simulink model "Residential_grid5"  (R2026a)
settings: Solver=VariableStepAuto  StopTime=365*24*3600
undefined symbols (not defined in the file): evCharge, load1, load2, load3, load4, load5, Solar, Wind
libraries: fl_lib x139, nesl_utility x68
(part 1 of 3)
settings Model: Creator=xiaos  LastModifiedBy=hiro
settings DebuggingCC: SaveWithParameterizedLinksMsg=none
settings SimscapeCC: SimscapeNominalValues="[{\"value\":\"1\",\"unit\":\"A\"},{\"value\":\"1\",\"unit\":\"bar\"},{\"value\":\"1\",\"unit\":\"cm^2\"},{\"value\":\"1\",\"unit\":\"cm^3/s\"},{\"value\":\"1\",\"unit\":\"kJ/kg\"},{\"value\":\"1\",\"unit\":\"kW\"},{\"value\":\"1\",\"unit\":\"l\"},{\"value\":\"1\",\"unit\":\"N\"},{\"value\":\"1\",\"unit\":\"N*m\"},{\"value\":\"1\",\"unit\":\"V\"}]"  SimscapeLogType=none  SimscapeLogDataHistory=5000.0

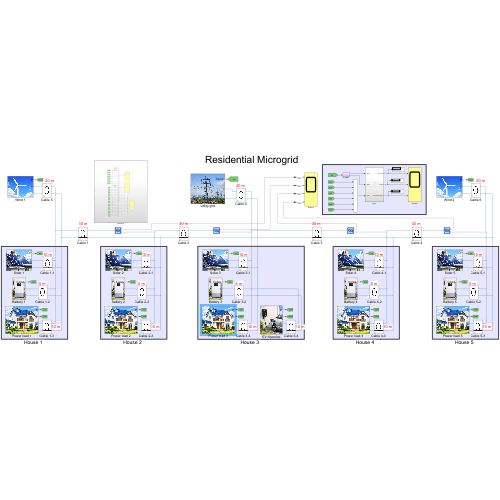
[thumbnail: Simulink's stored preview of the top-level diagram]
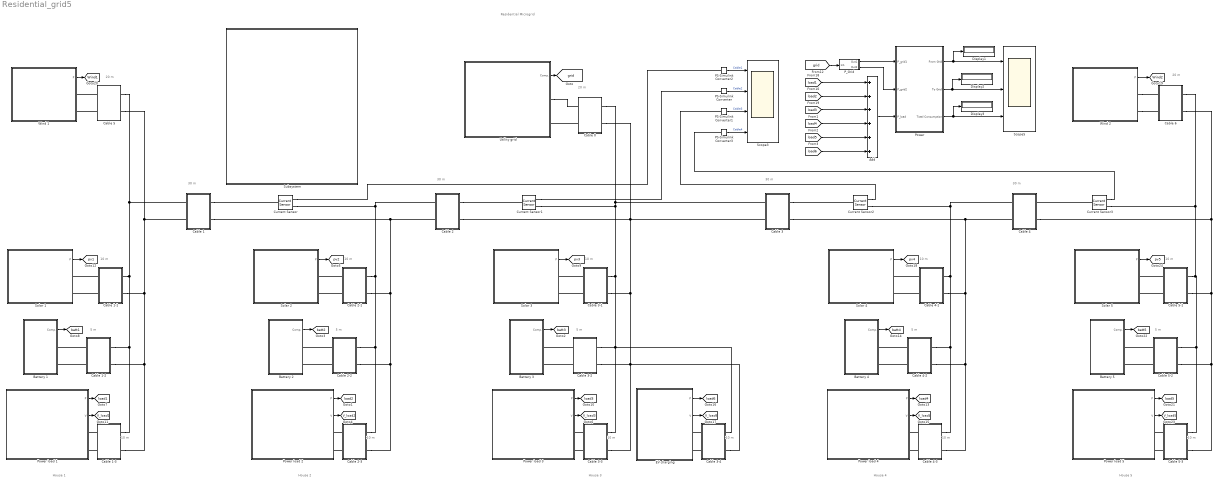
== system Residential_grid5 ==
  note: House 3
  note: House 2
  note: House 1
  note: House 4
  note: House 5
  note: Residential Microgrid
  note: 30 m
  note: 30 m
  note: 30 m
  note: 30 m
  note: 20 m
  note: 20 m
  note: 20 m
  note: 10 m
  note: 10 m
  note: 10 m
  note: 10 m
  note: 10 m
  note: 5 m
  note: 5 m
  note: 5 m
  note: 5 m
  note: 5 m
  note: 10 m
  note: 10 m
  note: 10 m
  note: 10 m
  note: 10 m
  note: 10 m
  Add : Sum  Inputs=++++++
  Battery 1 : Subsystem  mask{Cell=115, C_batt=20, SOC_Initial=50, R_int=75}
      mask prompts: Cell "Number of serial cells"; C_batt "Battery capacity (Ah)"; SOC_Initial "Initial SoC (%)"; R_int "Internal resistance (mΩ per Cell per Ah)"
      mask DialogControl DescTextVar Prompt: LiFePO4 Battery
      mask Display: image('Batt_1_4_1_1.png');
  Battery 2 : Subsystem  mask{Cell=115, C_batt=20, SOC_Initial=50, R_int=75}
      mask prompts: Cell "Number of serial cells"; C_batt "Battery capacity (Ah)"; SOC_Initial "Initial SoC (%)"; R_int "Internal resistance (mΩ per Cell per Ah)"
      mask DialogControl DescTextVar Prompt: LiFePO4 Battery
      mask Display: image('Batt_1_4_1_1.png');
  Battery 3 : Subsystem  mask{Cell=115, C_batt=20, SOC_Initial=50, R_int=75}
      mask prompts: Cell "Number of serial cells"; C_batt "Battery capacity (Ah)"; SOC_Initial "Initial SoC (%)"; R_int "Internal resistance (mΩ per Cell per Ah)"
      mask DialogControl DescTextVar Prompt: LiFePO4 Battery
      mask Display: image('Batt_1_4_1_1.png');
  Battery 4 : Subsystem  mask{Cell=115, C_batt=20, SOC_Initial=50, R_int=75}
      mask prompts: Cell "Number of serial cells"; C_batt "Battery capacity (Ah)"; SOC_Initial "Initial SoC (%)"; R_int "Internal resistance (mΩ per Cell per Ah)"
      mask DialogControl DescTextVar Prompt: LiFePO4 Battery
      mask Display: image('Batt_1_4_1_1.png');
  Battery 5 : Subsystem  mask{Cell=115, C_batt=20, SOC_Initial=50, R_int=75}
      mask prompts: Cell "Number of serial cells"; C_batt "Battery capacity (Ah)"; SOC_Initial "Initial SoC (%)"; R_int "Internal resistance (mΩ per Cell per Ah)"
      mask DialogControl DescTextVar Prompt: LiFePO4 Battery
      mask Display: image('Batt_1_4_1_1.png');
  Cable 0 : Subsystem  mask{intR=3.01, L=20, SQ=SQ,  rc,  Ampacity}
      mask prompts: intR "Conductor resistance: rc (Ω/km)"; L "Length: L (m)"; SQ "For reference: CV cable constants"
      mask TypeOptions SQ: SQ,  rc,  Ampacity | 2 (mm2),  12 (Ω/km),  28 (A) | 3.5 (mm2),  6.76 (Ω/km),  39 (A) | 5.5 (mm2),  4.34 (Ω/km),  52 (A) | 8 (mm2),  3.01 (Ω/km),   65 (A) | 14 (mm2),  1.71 (Ω/km),  91 (A) | 22 (mm2),  1.08 (Ω/km),  120 (A) | 38 (mm2),  0.626 (Ω/km),  170 (A) | 60 (mm2),  0.397 (Ω/km),  225 (A) | 100 (mm2),  0.239 (Ω/km),  310 (A) | 150 (mm2),  0.16 (Ω/km),  400 (A) | 200 (mm2),  0.121 (Ω/km),  485 (A) | 250 (mm2),  0.0985 (Ω/km),  560 (A) | 325 (mm2),  0.077 (Ω/km),  660 (A)
      mask DialogControl DescTextVar Prompt: 2-Core CV Cable
      mask Display: image('cable_1.png');
  Cable 1 : Subsystem  mask{intR=3.01, L=30, SQ=SQ,  rc,  Ampacity}
      mask prompts: intR "Conductor resistance: rc (Ω/km)"; L "Length: L (m)"; SQ "For reference: CV cable constants"
      mask TypeOptions SQ: SQ,  rc,  Ampacity | 2 (mm2),  12 (Ω/km),  28 (A) | 3.5 (mm2),  6.76 (Ω/km),  39 (A) | 5.5 (mm2),  4.34 (Ω/km),  52 (A) | 8 (mm2),  3.01 (Ω/km),   65 (A) | 14 (mm2),  1.71 (Ω/km),  91 (A) | 22 (mm2),  1.08 (Ω/km),  120 (A) | 38 (mm2),  0.626 (Ω/km),  170 (A) | 60 (mm2),  0.397 (Ω/km),  225 (A) | 100 (mm2),  0.239 (Ω/km),  310 (A) | 150 (mm2),  0.16 (Ω/km),  400 (A) | 200 (mm2),  0.121 (Ω/km),  485 (A) | 250 (mm2),  0.0985 (Ω/km),  560 (A) | 325 (mm2),  0.077 (Ω/km),  660 (A)
      mask DialogControl DescTextVar Prompt: 2-Core CV Cable
      mask Display: image('cable_2.png');
  Cable 1-1 : Subsystem  mask{intR=3.01, L=10, SQ=SQ,  rc,  Ampacity}
      mask prompts: intR "Conductor resistance: rc (Ω/km)"; L "Length: L (m)"; SQ "For reference: CV cable constants"
      mask TypeOptions SQ: SQ,  rc,  Ampacity | 2 (mm2),  12 (Ω/km),  28 (A) | 3.5 (mm2),  6.76 (Ω/km),  39 (A) | 5.5 (mm2),  4.34 (Ω/km),  52 (A) | 8 (mm2),  3.01 (Ω/km),   65 (A) | 14 (mm2),  1.71 (Ω/km),  91 (A) | 22 (mm2),  1.08 (Ω/km),  120 (A) | 38 (mm2),  0.626 (Ω/km),  170 (A) | 60 (mm2),  0.397 (Ω/km),  225 (A) | 100 (mm2),  0.239 (Ω/km),  310 (A) | 150 (mm2),  0.16 (Ω/km),  400 (A) | 200 (mm2),  0.121 (Ω/km),  485 (A) | 250 (mm2),  0.0985 (Ω/km),  560 (A) | 325 (mm2),  0.077 (Ω/km),  660 (A)
      mask DialogControl DescTextVar Prompt: 2-Core CV Cable
      mask Display: image('cable_9.png');
  Cable 1-2 : Subsystem  mask{intR=3.01, L=5, SQ=SQ,  rc,  Ampacity}
      mask prompts: intR "Conductor resistance: rc (Ω/km)"; L "Length: L (m)"; SQ "For reference: CV cable constants"
      mask TypeOptions SQ: SQ,  rc,  Ampacity | 2 (mm2),  12 (Ω/km),  28 (A) | 3.5 (mm2),  6.76 (Ω/km),  39 (A) | 5.5 (mm2),  4.34 (Ω/km),  52 (A) | 8 (mm2),  3.01 (Ω/km),   65 (A) | 14 (mm2),  1.71 (Ω/km),  91 (A) | 22 (mm2),  1.08 (Ω/km),  120 (A) | 38 (mm2),  0.626 (Ω/km),  170 (A) | 60 (mm2),  0.397 (Ω/km),  225 (A) | 100 (mm2),  0.239 (Ω/km),  310 (A) | 150 (mm2),  0.16 (Ω/km),  400 (A) | 200 (mm2),  0.121 (Ω/km),  485 (A) | 250 (mm2),  0.0985 (Ω/km),  560 (A) | 325 (mm2),  0.077 (Ω/km),  660 (A)
      mask DialogControl DescTextVar Prompt: 2-Core CV Cable
      mask Display: image('cable_7.png');
  Cable 1-3 : Subsystem  mask{intR=3.01, L=10, SQ=SQ,  rc,  Ampacity}
      mask prompts: intR "Conductor resistance: rc (Ω/km)"; L "Length: L (m)"; SQ "For reference: CV cable constants"
      mask TypeOptions SQ: SQ,  rc,  Ampacity | 2 (mm2),  12 (Ω/km),  28 (A) | 3.5 (mm2),  6.76 (Ω/km),  39 (A) | 5.5 (mm2),  4.34 (Ω/km),  52 (A) | 8 (mm2),  3.01 (Ω/km),   65 (A) | 14 (mm2),  1.71 (Ω/km),  91 (A) | 22 (mm2),  1.08 (Ω/km),  120 (A) | 38 (mm2),  0.626 (Ω/km),  170 (A) | 60 (mm2),  0.397 (Ω/km),  225 (A) | 100 (mm2),  0.239 (Ω/km),  310 (A) | 150 (mm2),  0.16 (Ω/km),  400 (A) | 200 (mm2),  0.121 (Ω/km),  485 (A) | 250 (mm2),  0.0985 (Ω/km),  560 (A) | 325 (mm2),  0.077 (Ω/km),  660 (A)
      mask DialogControl DescTextVar Prompt: 2-Core CV Cable
      mask Display: image('cable_8.png');
  Cable 2 : Subsystem  mask{intR=3.01, L=30, SQ=SQ,  rc,  Ampacity}
      mask prompts: intR "Conductor resistance: rc (Ω/km)"; L "Length: L (m)"; SQ "For reference: CV cable constants"
      mask TypeOptions SQ: SQ,  rc,  Ampacity | 2 (mm2),  12 (Ω/km),  28 (A) | 3.5 (mm2),  6.76 (Ω/km),  39 (A) | 5.5 (mm2),  4.34 (Ω/km),  52 (A) | 8 (mm2),  3.01 (Ω/km),   65 (A) | 14 (mm2),  1.71 (Ω/km),  91 (A) | 22 (mm2),  1.08 (Ω/km),  120 (A) | 38 (mm2),  0.626 (Ω/km),  170 (A) | 60 (mm2),  0.397 (Ω/km),  225 (A) | 100 (mm2),  0.239 (Ω/km),  310 (A) | 150 (mm2),  0.16 (Ω/km),  400 (A) | 200 (mm2),  0.121 (Ω/km),  485 (A) | 250 (mm2),  0.0985 (Ω/km),  560 (A) | 325 (mm2),  0.077 (Ω/km),  660 (A)
      mask DialogControl DescTextVar Prompt: 2-Core CV Cable
      mask Display: image('cable_3.png');
  Cable 2-1 : Subsystem  mask{intR=3.01, L=10, SQ=SQ,  rc,  Ampacity}
      mask prompts: intR "Conductor resistance: rc (Ω/km)"; L "Length: L (m)"; SQ "For reference: CV cable constants"
      mask TypeOptions SQ: SQ,  rc,  Ampacity | 2 (mm2),  12 (Ω/km),  28 (A) | 3.5 (mm2),  6.76 (Ω/km),  39 (A) | 5.5 (mm2),  4.34 (Ω/km),  52 (A) | 8 (mm2),  3.01 (Ω/km),   65 (A) | 14 (mm2),  1.71 (Ω/km),  91 (A) | 22 (mm2),  1.08 (Ω/km),  120 (A) | 38 (mm2),  0.626 (Ω/km),  170 (A) | 60 (mm2),  0.397 (Ω/km),  225 (A) | 100 (mm2),  0.239 (Ω/km),  310 (A) | 150 (mm2),  0.16 (Ω/km),  400 (A) | 200 (mm2),  0.121 (Ω/km),  485 (A) | 250 (mm2),  0.0985 (Ω/km),  560 (A) | 325 (mm2),  0.077 (Ω/km),  660 (A)
      mask DialogControl DescTextVar Prompt: 2-Core CV Cable
      mask Display: image('cable_9.png');
  Cable 2-2 : Subsystem  mask{intR=3.01, L=5, SQ=SQ,  rc,  Ampacity}
      mask prompts: intR "Conductor resistance: rc (Ω/km)"; L "Length: L (m)"; SQ "For reference: CV cable constants"
      mask TypeOptions SQ: SQ,  rc,  Ampacity | 2 (mm2),  12 (Ω/km),  28 (A) | 3.5 (mm2),  6.76 (Ω/km),  39 (A) | 5.5 (mm2),  4.34 (Ω/km),  52 (A) | 8 (mm2),  3.01 (Ω/km),   65 (A) | 14 (mm2),  1.71 (Ω/km),  91 (A) | 22 (mm2),  1.08 (Ω/km),  120 (A) | 38 (mm2),  0.626 (Ω/km),  170 (A) | 60 (mm2),  0.397 (Ω/km),  225 (A) | 100 (mm2),  0.239 (Ω/km),  310 (A) | 150 (mm2),  0.16 (Ω/km),  400 (A) | 200 (mm2),  0.121 (Ω/km),  485 (A) | 250 (mm2),  0.0985 (Ω/km),  560 (A) | 325 (mm2),  0.077 (Ω/km),  660 (A)
      mask DialogControl DescTextVar Prompt: 2-Core CV Cable
      mask Display: image('cable_7.png');
  Cable 2-3 : Subsystem  mask{intR=3.01, L=10, SQ=SQ,  rc,  Ampacity}
      mask prompts: intR "Conductor resistance: rc (Ω/km)"; L "Length: L (m)"; SQ "For reference: CV cable constants"
      mask TypeOptions SQ: SQ,  rc,  Ampacity | 2 (mm2),  12 (Ω/km),  28 (A) | 3.5 (mm2),  6.76 (Ω/km),  39 (A) | 5.5 (mm2),  4.34 (Ω/km),  52 (A) | 8 (mm2),  3.01 (Ω/km),   65 (A) | 14 (mm2),  1.71 (Ω/km),  91 (A) | 22 (mm2),  1.08 (Ω/km),  120 (A) | 38 (mm2),  0.626 (Ω/km),  170 (A) | 60 (mm2),  0.397 (Ω/km),  225 (A) | 100 (mm2),  0.239 (Ω/km),  310 (A) | 150 (mm2),  0.16 (Ω/km),  400 (A) | 200 (mm2),  0.121 (Ω/km),  485 (A) | 250 (mm2),  0.0985 (Ω/km),  560 (A) | 325 (mm2),  0.077 (Ω/km),  660 (A)
      mask DialogControl DescTextVar Prompt: 2-Core CV Cable
      mask Display: image('cable_8.png');
  Cable 3 : Subsystem  mask{intR=3.01, L=30, SQ=SQ,  rc,  Ampacity}
      mask prompts: intR "Conductor resistance: rc (Ω/km)"; L "Length: L (m)"; SQ "For reference: CV cable constants"
      mask TypeOptions SQ: SQ,  rc,  Ampacity | 2 (mm2),  12 (Ω/km),  28 (A) | 3.5 (mm2),  6.76 (Ω/km),  39 (A) | 5.5 (mm2),  4.34 (Ω/km),  52 (A) | 8 (mm2),  3.01 (Ω/km),   65 (A) | 14 (mm2),  1.71 (Ω/km),  91 (A) | 22 (mm2),  1.08 (Ω/km),  120 (A) | 38 (mm2),  0.626 (Ω/km),  170 (A) | 60 (mm2),  0.397 (Ω/km),  225 (A) | 100 (mm2),  0.239 (Ω/km),  310 (A) | 150 (mm2),  0.16 (Ω/km),  400 (A) | 200 (mm2),  0.121 (Ω/km),  485 (A) | 250 (mm2),  0.0985 (Ω/km),  560 (A) | 325 (mm2),  0.077 (Ω/km),  660 (A)
      mask DialogControl DescTextVar Prompt: 2-Core CV Cable
      mask Display: image('cable_4.png');
  Cable 3-1 : Subsystem  mask{intR=3.01, L=10, SQ=SQ,  rc,  Ampacity}
      mask prompts: intR "Conductor resistance: rc (Ω/km)"; L "Length: L (m)"; SQ "For reference: CV cable constants"
      mask TypeOptions SQ: SQ,  rc,  Ampacity | 2 (mm2),  12 (Ω/km),  28 (A) | 3.5 (mm2),  6.76 (Ω/km),  39 (A) | 5.5 (mm2),  4.34 (Ω/km),  52 (A) | 8 (mm2),  3.01 (Ω/km),   65 (A) | 14 (mm2),  1.71 (Ω/km),  91 (A) | 22 (mm2),  1.08 (Ω/km),  120 (A) | 38 (mm2),  0.626 (Ω/km),  170 (A) | 60 (mm2),  0.397 (Ω/km),  225 (A) | 100 (mm2),  0.239 (Ω/km),  310 (A) | 150 (mm2),  0.16 (Ω/km),  400 (A) | 200 (mm2),  0.121 (Ω/km),  485 (A) | 250 (mm2),  0.0985 (Ω/km),  560 (A) | 325 (mm2),  0.077 (Ω/km),  660 (A)
      mask DialogControl DescTextVar Prompt: 2-Core CV Cable
      mask Display: image('cable_9.png');
  Cable 3-2 : Subsystem  mask{intR=3.01, L=5, SQ=SQ,  rc,  Ampacity}
      mask prompts: intR "Conductor resistance: rc (Ω/km)"; L "Length: L (m)"; SQ "For reference: CV cable constants"
      mask TypeOptions SQ: SQ,  rc,  Ampacity | 2 (mm2),  12 (Ω/km),  28 (A) | 3.5 (mm2),  6.76 (Ω/km),  39 (A) | 5.5 (mm2),  4.34 (Ω/km),  52 (A) | 8 (mm2),  3.01 (Ω/km),   65 (A) | 14 (mm2),  1.71 (Ω/km),  91 (A) | 22 (mm2),  1.08 (Ω/km),  120 (A) | 38 (mm2),  0.626 (Ω/km),  170 (A) | 60 (mm2),  0.397 (Ω/km),  225 (A) | 100 (mm2),  0.239 (Ω/km),  310 (A) | 150 (mm2),  0.16 (Ω/km),  400 (A) | 200 (mm2),  0.121 (Ω/km),  485 (A) | 250 (mm2),  0.0985 (Ω/km),  560 (A) | 325 (mm2),  0.077 (Ω/km),  660 (A)
      mask DialogControl DescTextVar Prompt: 2-Core CV Cable
      mask Display: image('cable_7.png');
  Cable 3-3 : Subsystem  mask{intR=3.01, L=10, SQ=SQ,  rc,  Ampacity}
      mask prompts: intR "Conductor resistance: rc (Ω/km)"; L "Length: L (m)"; SQ "For reference: CV cable constants"
      mask TypeOptions SQ: SQ,  rc,  Ampacity | 2 (mm2),  12 (Ω/km),  28 (A) | 3.5 (mm2),  6.76 (Ω/km),  39 (A) | 5.5 (mm2),  4.34 (Ω/km),  52 (A) | 8 (mm2),  3.01 (Ω/km),   65 (A) | 14 (mm2),  1.71 (Ω/km),  91 (A) | 22 (mm2),  1.08 (Ω/km),  120 (A) | 38 (mm2),  0.626 (Ω/km),  170 (A) | 60 (mm2),  0.397 (Ω/km),  225 (A) | 100 (mm2),  0.239 (Ω/km),  310 (A) | 150 (mm2),  0.16 (Ω/km),  400 (A) | 200 (mm2),  0.121 (Ω/km),  485 (A) | 250 (mm2),  0.0985 (Ω/km),  560 (A) | 325 (mm2),  0.077 (Ω/km),  660 (A)
      mask DialogControl DescTextVar Prompt: 2-Core CV Cable
      mask Display: image('cable_8.png');
  Cable 3-4 : Subsystem  mask{intR=3.01, L=10, SQ=SQ,  rc,  Ampacity}
      mask prompts: intR "Conductor resistance: rc (Ω/km)"; L "Length: L (m)"; SQ "For reference: CV cable constants"
      mask TypeOptions SQ: SQ,  rc,  Ampacity | 2 (mm2),  12 (Ω/km),  28 (A) | 3.5 (mm2),  6.76 (Ω/km),  39 (A) | 5.5 (mm2),  4.34 (Ω/km),  52 (A) | 8 (mm2),  3.01 (Ω/km),   65 (A) | 14 (mm2),  1.71 (Ω/km),  91 (A) | 22 (mm2),  1.08 (Ω/km),  120 (A) | 38 (mm2),  0.626 (Ω/km),  170 (A) | 60 (mm2),  0.397 (Ω/km),  225 (A) | 100 (mm2),  0.239 (Ω/km),  310 (A) | 150 (mm2),  0.16 (Ω/km),  400 (A) | 200 (mm2),  0.121 (Ω/km),  485 (A) | 250 (mm2),  0.0985 (Ω/km),  560 (A) | 325 (mm2),  0.077 (Ω/km),  660 (A)
      mask DialogControl DescTextVar Prompt: 2-Core CV Cable
      mask Display: image('cable_8.png');
  Cable 4 : Subsystem  mask{intR=3.01, L=30, SQ=SQ,  rc,  Ampacity}
      mask prompts: intR "Conductor resistance: rc (Ω/km)"; L "Length: L (m)"; SQ "For reference: CV cable constants"
      mask TypeOptions SQ: SQ,  rc,  Ampacity | 2 (mm2),  12 (Ω/km),  28 (A) | 3.5 (mm2),  6.76 (Ω/km),  39 (A) | 5.5 (mm2),  4.34 (Ω/km),  52 (A) | 8 (mm2),  3.01 (Ω/km),   65 (A) | 14 (mm2),  1.71 (Ω/km),  91 (A) | 22 (mm2),  1.08 (Ω/km),  120 (A) | 38 (mm2),  0.626 (Ω/km),  170 (A) | 60 (mm2),  0.397 (Ω/km),  225 (A) | 100 (mm2),  0.239 (Ω/km),  310 (A) | 150 (mm2),  0.16 (Ω/km),  400 (A) | 200 (mm2),  0.121 (Ω/km),  485 (A) | 250 (mm2),  0.0985 (Ω/km),  560 (A) | 325 (mm2),  0.077 (Ω/km),  660 (A)
      mask DialogControl DescTextVar Prompt: 2-Core CV Cable
      mask Display: image('cable_5.png');
  Cable 4-1 : Subsystem  mask{intR=3.01, L=10, SQ=SQ,  rc,  Ampacity}
      mask prompts: intR "Conductor resistance: rc (Ω/km)"; L "Length: L (m)"; SQ "For reference: CV cable constants"
      mask TypeOptions SQ: SQ,  rc,  Ampacity | 2 (mm2),  12 (Ω/km),  28 (A) | 3.5 (mm2),  6.76 (Ω/km),  39 (A) | 5.5 (mm2),  4.34 (Ω/km),  52 (A) | 8 (mm2),  3.01 (Ω/km),   65 (A) | 14 (mm2),  1.71 (Ω/km),  91 (A) | 22 (mm2),  1.08 (Ω/km),  120 (A) | 38 (mm2),  0.626 (Ω/km),  170 (A) | 60 (mm2),  0.397 (Ω/km),  225 (A) | 100 (mm2),  0.239 (Ω/km),  310 (A) | 150 (mm2),  0.16 (Ω/km),  400 (A) | 200 (mm2),  0.121 (Ω/km),  485 (A) | 250 (mm2),  0.0985 (Ω/km),  560 (A) | 325 (mm2),  0.077 (Ω/km),  660 (A)
      mask DialogControl DescTextVar Prompt: 2-Core CV Cable
      mask Display: image('cable_9.png');
  Cable 4-2 : Subsystem  mask{intR=3.01, L=5, SQ=SQ,  rc,  Ampacity}
      mask prompts: intR "Conductor resistance: rc (Ω/km)"; L "Length: L (m)"; SQ "For reference: CV cable constants"
      mask TypeOptions SQ: SQ,  rc,  Ampacity | 2 (mm2),  12 (Ω/km),  28 (A) | 3.5 (mm2),  6.76 (Ω/km),  39 (A) | 5.5 (mm2),  4.34 (Ω/km),  52 (A) | 8 (mm2),  3.01 (Ω/km),   65 (A) | 14 (mm2),  1.71 (Ω/km),  91 (A) | 22 (mm2),  1.08 (Ω/km),  120 (A) | 38 (mm2),  0.626 (Ω/km),  170 (A) | 60 (mm2),  0.397 (Ω/km),  225 (A) | 100 (mm2),  0.239 (Ω/km),  310 (A) | 150 (mm2),  0.16 (Ω/km),  400 (A) | 200 (mm2),  0.121 (Ω/km),  485 (A) | 250 (mm2),  0.0985 (Ω/km),  560 (A) | 325 (mm2),  0.077 (Ω/km),  660 (A)
      mask DialogControl DescTextVar Prompt: 2-Core CV Cable
      mask Display: image('cable_7.png');
  Cable 4-3 : Subsystem  mask{intR=3.01, L=10, SQ=SQ,  rc,  Ampacity}
      mask prompts: intR "Conductor resistance: rc (Ω/km)"; L "Length: L (m)"; SQ "For reference: CV cable constants"
      mask TypeOptions SQ: SQ,  rc,  Ampacity | 2 (mm2),  12 (Ω/km),  28 (A) | 3.5 (mm2),  6.76 (Ω/km),  39 (A) | 5.5 (mm2),  4.34 (Ω/km),  52 (A) | 8 (mm2),  3.01 (Ω/km),   65 (A) | 14 (mm2),  1.71 (Ω/km),  91 (A) | 22 (mm2),  1.08 (Ω/km),  120 (A) | 38 (mm2),  0.626 (Ω/km),  170 (A) | 60 (mm2),  0.397 (Ω/km),  225 (A) | 100 (mm2),  0.239 (Ω/km),  310 (A) | 150 (mm2),  0.16 (Ω/km),  400 (A) | 200 (mm2),  0.121 (Ω/km),  485 (A) | 250 (mm2),  0.0985 (Ω/km),  560 (A) | 325 (mm2),  0.077 (Ω/km),  660 (A)
      mask DialogControl DescTextVar Prompt: 2-Core CV Cable
      mask Display: image('cable_8.png');
  Cable 5 : Subsystem  mask{intR=3.01, L=20, SQ=SQ,  rc,  Ampacity}
      mask prompts: intR "Conductor resistance: rc (Ω/km)"; L "Length: L (m)"; SQ "For reference: CV cable constants"
      mask TypeOptions SQ: SQ,  rc,  Ampacity | 2 (mm2),  12 (Ω/km),  28 (A) | 3.5 (mm2),  6.76 (Ω/km),  39 (A) | 5.5 (mm2),  4.34 (Ω/km),  52 (A) | 8 (mm2),  3.01 (Ω/km),   65 (A) | 14 (mm2),  1.71 (Ω/km),  91 (A) | 22 (mm2),  1.08 (Ω/km),  120 (A) | 38 (mm2),  0.626 (Ω/km),  170 (A) | 60 (mm2),  0.397 (Ω/km),  225 (A) | 100 (mm2),  0.239 (Ω/km),  310 (A) | 150 (mm2),  0.16 (Ω/km),  400 (A) | 200 (mm2),  0.121 (Ω/km),  485 (A) | 250 (mm2),  0.0985 (Ω/km),  560 (A) | 325 (mm2),  0.077 (Ω/km),  660 (A)
      mask DialogControl DescTextVar Prompt: 2-Core CV Cable
      mask Display: image('cable_6.png');
  Cable 5-1 : Subsystem  mask{intR=3.01, L=10, SQ=SQ,  rc,  Ampacity}
      mask prompts: intR "Conductor resistance: rc (Ω/km)"; L "Length: L (m)"; SQ "For reference: CV cable constants"
      mask TypeOptions SQ: SQ,  rc,  Ampacity | 2 (mm2),  12 (Ω/km),  28 (A) | 3.5 (mm2),  6.76 (Ω/km),  39 (A) | 5.5 (mm2),  4.34 (Ω/km),  52 (A) | 8 (mm2),  3.01 (Ω/km),   65 (A) | 14 (mm2),  1.71 (Ω/km),  91 (A) | 22 (mm2),  1.08 (Ω/km),  120 (A) | 38 (mm2),  0.626 (Ω/km),  170 (A) | 60 (mm2),  0.397 (Ω/km),  225 (A) | 100 (mm2),  0.239 (Ω/km),  310 (A) | 150 (mm2),  0.16 (Ω/km),  400 (A) | 200 (mm2),  0.121 (Ω/km),  485 (A) | 250 (mm2),  0.0985 (Ω/km),  560 (A) | 325 (mm2),  0.077 (Ω/km),  660 (A)
      mask DialogControl DescTextVar Prompt: 2-Core CV Cable
      mask Display: image('cable_9.png');
  Cable 5-2 : Subsystem  mask{intR=3.01, L=5, SQ=SQ,  rc,  Ampacity}
      mask prompts: intR "Conductor resistance: rc (Ω/km)"; L "Length: L (m)"; SQ "For reference: CV cable constants"
      mask TypeOptions SQ: SQ,  rc,  Ampacity | 2 (mm2),  12 (Ω/km),  28 (A) | 3.5 (mm2),  6.76 (Ω/km),  39 (A) | 5.5 (mm2),  4.34 (Ω/km),  52 (A) | 8 (mm2),  3.01 (Ω/km),   65 (A) | 14 (mm2),  1.71 (Ω/km),  91 (A) | 22 (mm2),  1.08 (Ω/km),  120 (A) | 38 (mm2),  0.626 (Ω/km),  170 (A) | 60 (mm2),  0.397 (Ω/km),  225 (A) | 100 (mm2),  0.239 (Ω/km),  310 (A) | 150 (mm2),  0.16 (Ω/km),  400 (A) | 200 (mm2),  0.121 (Ω/km),  485 (A) | 250 (mm2),  0.0985 (Ω/km),  560 (A) | 325 (mm2),  0.077 (Ω/km),  660 (A)
      mask DialogControl DescTextVar Prompt: 2-Core CV Cable
      mask Display: image('cable_7.png');
  Cable 5-3 : Subsystem  mask{intR=3.01, L=10, SQ=SQ,  rc,  Ampacity}
      mask prompts: intR "Conductor resistance: rc (Ω/km)"; L "Length: L (m)"; SQ "For reference: CV cable constants"
      mask TypeOptions SQ: SQ,  rc,  Ampacity | 2 (mm2),  12 (Ω/km),  28 (A) | 3.5 (mm2),  6.76 (Ω/km),  39 (A) | 5.5 (mm2),  4.34 (Ω/km),  52 (A) | 8 (mm2),  3.01 (Ω/km),   65 (A) | 14 (mm2),  1.71 (Ω/km),  91 (A) | 22 (mm2),  1.08 (Ω/km),  120 (A) | 38 (mm2),  0.626 (Ω/km),  170 (A) | 60 (mm2),  0.397 (Ω/km),  225 (A) | 100 (mm2),  0.239 (Ω/km),  310 (A) | 150 (mm2),  0.16 (Ω/km),  400 (A) | 200 (mm2),  0.121 (Ω/km),  485 (A) | 250 (mm2),  0.0985 (Ω/km),  560 (A) | 325 (mm2),  0.077 (Ω/km),  660 (A)
      mask DialogControl DescTextVar Prompt: 2-Core CV Cable
      mask Display: image('cable_8.png');
  Cable 6 : Subsystem  mask{intR=3.01, L=20, SQ=SQ,  rc,  Ampacity}
      mask prompts: intR "Conductor resistance: rc (Ω/km)"; L "Length: L (m)"; SQ "For reference: CV cable constants"
      mask TypeOptions SQ: SQ,  rc,  Ampacity | 2 (mm2),  12 (Ω/km),  28 (A) | 3.5 (mm2),  6.76 (Ω/km),  39 (A) | 5.5 (mm2),  4.34 (Ω/km),  52 (A) | 8 (mm2),  3.01 (Ω/km),   65 (A) | 14 (mm2),  1.71 (Ω/km),  91 (A) | 22 (mm2),  1.08 (Ω/km),  120 (A) | 38 (mm2),  0.626 (Ω/km),  170 (A) | 60 (mm2),  0.397 (Ω/km),  225 (A) | 100 (mm2),  0.239 (Ω/km),  310 (A) | 150 (mm2),  0.16 (Ω/km),  400 (A) | 200 (mm2),  0.121 (Ω/km),  485 (A) | 250 (mm2),  0.0985 (Ω/km),  560 (A) | 325 (mm2),  0.077 (Ω/km),  660 (A)
      mask DialogControl DescTextVar Prompt: 2-Core CV Cable
      mask Display: image('cable_6.png');
  Current Sensor{,1..3} (4 alike) : fl_lib/Electrical/Electrical Sensors/Current Sensor
  Display1 : Display
  Display2 : Display
  Display3 : Display
  EV charging : Subsystem  mask{data=evCharge, timestep=[0:1:24*3600*365-1]}
      mask prompts: data "Power consumption data"
      mask DialogControl DescGroupVar Prompt: EV Charging
      mask Display: image('EV_Charge_1.png');
  PS-Simulink Converter{,1..3} (4 alike) : nesl_utility/PS-Simulink Converter  PhysicalDomain=network_engine_domain  SubClassName=ps_output  LeftPortType=input  RightPortType=output  PseudoPeriodic=off  Frequencies=[]  VectorFormat=inherit  Unit=inherit  AffineConversion=off
  P_Grid : Subsystem
  Power : Subsystem
  Power load 1 : Subsystem  mask{data=load1, timestep=[0:1:24*3600*365-1]}
      mask prompts: data "Power consumption data"
      mask DialogControl DescGroupVar Prompt: Power Load
      mask Display: image('House_1.png');
  Power load 2 : Subsystem  mask{data=load2, timestep=[0:1:24*3600*365-1]}
      mask prompts: data "Power consumption data"
      mask DialogControl DescGroupVar Prompt: Power Load
      mask Display: image('House_1.png');
  Power load 3 : Subsystem  mask{data=load3, timestep=[0:1:24*3600*365-1]}
      mask prompts: data "Power consumption data"
      mask DialogControl DescGroupVar Prompt: Power Load
      mask Display: image('House_1.png');
  Power load 4 : Subsystem  mask{data=load4, timestep=[0:1:24*3600*365-1]}
      mask prompts: data "Power consumption data"
      mask DialogControl DescGroupVar Prompt: Power Load
      mask Display: image('House_1.png');
  Power load 5 : Subsystem  mask{data=load5, timestep=[0:1:24*3600*365-1]}
      mask prompts: data "Power consumption data"
      mask DialogControl DescGroupVar Prompt: Power Load
      mask Display: image('House_1.png');
  Scope3 : Scope  NumInputPorts=4
      settings: ActiveDisplayYMinimum=-18.216451642812157  ActiveDisplayYMaximum=17.414891932696229  YLabel=Current (A)  DataLoggingDecimation=60
  Scope5 : Scope  NumInputPorts=3
      settings: ActiveDisplayYMinimum=-1.4420520970231628E+8  ActiveDisplayYMaximum=9.0945805640393951E+10  YLabel=Accumulated Power (W Sec)  DataLoggingDecimation=60  DataLoggingVariableName=ScopeData17
  Solar 1 : Subsystem  mask{POA=Solar.POA(:,2), Coef=Solar.Coef(:,2), kw=3.5, eff=100, V_Limit=400, Gain=100, timestep=[0:1:24*3600*365-1]}
      mask prompts: POA "Panel of array irradiance: POA"; Coef "Temperature correction coefficient"; kw "Rated output power (kW)"; eff "Location-based efficiency (%)"; V_Limit "Output curtailment start voltage (V)"; Gain "Overvoltage suppression gain (typ. 500)"
      mask DialogControl DescTextVar Prompt: Solar Power System
      mask Display: image('PV_1.png');
  Solar 2 : Subsystem  mask{POA=Solar.POA(:,5), Coef=Solar.Coef(:,5), kw=3.5, eff=100, V_Limit=400, Gain=100, timestep=[0:1:24*3600*365-1]}
      mask prompts: POA "Panel of array irradiance: POA"; Coef "Temperature correction coefficient"; kw "Rated output power (kW)"; eff "Location-based efficiency (%)"; V_Limit "Output curtailment start voltage (V)"; Gain "Overvoltage suppression gain (typ. 500)"
      mask DialogControl DescTextVar Prompt: Solar Power System
      mask Display: image('PV_1.png');
  Solar 3 : Subsystem  mask{POA=Solar.POA(:,1), Coef=Solar.Coef(:,1), kw=3.5, eff=100, V_Limit=400, Gain=100, timestep=[0:1:24*3600*365-1]}
      mask prompts: POA "Panel of array irradiance: POA"; Coef "Temperature correction coefficient"; kw "Rated output power (kW)"; eff "Location-based efficiency (%)"; V_Limit "Output curtailment start voltage (V)"; Gain "Overvoltage suppression gain (typ. 500)"
      mask DialogControl DescTextVar Prompt: Solar Power System
      mask Display: image('PV_1.png');
  Solar 4 : Subsystem  mask{POA=Solar.POA(:,5), Coef=Solar.Coef(:,5), kw=3.5, eff=100, V_Limit=400, Gain=100, timestep=[0:1:24*3600*365-1]}
      mask prompts: POA "Panel of array irradiance: POA"; Coef "Temperature correction coefficient"; kw "Rated output power (kW)"; eff "Location-based efficiency (%)"; V_Limit "Output curtailment start voltage (V)"; Gain "Overvoltage suppression gain (typ. 500)"
      mask DialogControl DescTextVar Prompt: Solar Power System
      mask Display: image('PV_1.png');
  Solar 5 : Subsystem  mask{POA=Solar.POA(:,8), Coef=Solar.Coef(:,8), kw=3.5, eff=100, V_Limit=400, Gain=100, timestep=[0:1:24*3600*365-1]}
      mask prompts: POA "Panel of array irradiance: POA"; Coef "Temperature correction coefficient"; kw "Rated output power (kW)"; eff "Location-based efficiency (%)"; V_Limit "Output curtailment start voltage (V)"; Gain "Overvoltage suppression gain (typ. 500)"
      mask DialogControl DescTextVar Prompt: Solar Power System
      mask Display: image('PV_1.png');
  Subsystem : Subsystem
  Utility grid : Subsystem  mask{dcbus=380, on=20, off=10, current=25}
      mask prompts: dcbus "DC-bus voltage (V)"; on "Grid‑assist ON threshold window (±V)"; off "Grid‑assist OFF threshold window (±V)"; current "Grid import/export current (A)"
      mask DialogControl DescTextVar Prompt: Power exchange with the utility grid
      mask Display: image('Grid_1.png');
  Wind 1 : Subsystem  mask{P_rate=1000, v_rate=10, v_cutin=2, v_cutout=25, V_Limit=400, Gain=100, timestep=[0:1:24*3600*365-1]}
      mask prompts: P_rate "Rated power generation (W)"; v_rate "Rated wind speed (m/s)"; v_cutin "Cut-in wind speed (m/s)"; v_cutout "Cut-out wind speed (m/s)"; V_Limit "Output curtailment start voltage (V)"; Gain "Overvoltage suppression gain (typ. 500)"
      mask DialogControl DescTextVar Prompt: Wind Power System
      mask Display: image('Windmill_1.png');
  Wind 2 : Subsystem  mask{P_rate=1000, v_rate=10, v_cutin=2, v_cutout=25, V_Limit=400, Gain=100, timestep=[0:1:24*3600*365-1]}
      mask prompts: P_rate "Rated power generation (W)"; v_rate "Rated wind speed (m/s)"; v_cutin "Cut-in wind speed (m/s)"; v_cutout "Cut-out wind speed (m/s)"; V_Limit "Output curtailment start voltage (V)"; Gain "Overvoltage suppression gain (typ. 500)"
      mask DialogControl DescTextVar Prompt: Wind Power System
      mask Display: image('Windmill_1_1.png');
  tag scope: V_load1=global, V_load2=global, V_load3=global, V_load4=global, V_load5=global, V_load6=global, Wind1=global, Wind2=global, batt1=global, batt2=global, batt3=global, batt4=global, batt5=global, grid=global, load1=global, load2=global, load3=global, load4=global, load5=global, load6=global, pv1=global, pv2=global, pv3=global, pv4=global, pv5=global
  wires:
  Power/3(Total Consumption) -> Display3/1, Scope5/3
  [load4] -> Add/4
  P_Grid/2(Out2) -> Power/2(P_grid2)
  [load2] -> Add/2
  Add/1 -> Power/3(P_load)
  [load5] -> Add/5
  Power/2(To Grid) -> Display2/1, Scope5/2
  P_Grid/1(Out1) -> Power/1(P_grid1)
  [load1] -> Add/1
  [load3] -> Add/3
  [grid] -> P_Grid/1(In1)
  Power/1(From Grid) -> Display1/1, Scope5/1
  EV charging/1(P) -> [load6]
  EV charging/2(V) -> [V_load6]
  Utility grid/1(Comp.) -> [grid]
  Wind 1/1(P) -> [Wind1]
  Wind 2/1(P) -> [Wind2]
  Power load 3/2(V) -> [V_load3]
  Battery 3/1(Comp.) -> [batt3]
  Solar 3/1(P) -> [pv3]
  Power load 3/1(P) -> [load3]
  Power load 2/2(V) -> [V_load2]
  Battery 2/1(Comp.) -> [batt2]
  Solar 2/1(P) -> [pv2]
  Power load 2/1(P) -> [load2]
  Power load 1/2(V) -> [V_load1]
  Battery 1/1(Comp.) -> [batt1]
  Solar 1/1(P) -> [pv1]
  Power load 1/1(P) -> [load1]
  Power load 4/2(V) -> [V_load4]
  Battery 4/1(Comp.) -> [batt4]
  Solar 4/1(P) -> [pv4]
  Power load 4/1(P) -> [load4]
  Power load 5/2(V) -> [V_load5]
  Battery 5/1(Comp.) -> [batt5]
  Solar 5/1(P) -> [pv5]
  Power load 5/1(P) -> [load5]
  PS-Simulink Converter2/1 -> Scope3/1  "Cable1"
  PS-Simulink Converter/1 -> Scope3/2  "Cable2"
  PS-Simulink Converter1/1 -> Scope3/3  "Cable3"
  PS-Simulink Converter3/1 -> Scope3/4  "Cable4"
  [load6] -> Add/6
  connections:
  Cable 1/RConn1 -- Current Sensor/LConn1
  Cable 2/RConn1 -- Current Sensor1/LConn1
  Cable 3-1/LConn1 -- Solar 3/RConn1
  Cable 3-1/LConn2 -- Solar 3/RConn2
  Cable 3-3/LConn1 -- Power load 3/RConn1
  Cable 3-2/LConn2 -- Battery 3/RConn2
  Cable 3-3/LConn2 -- Power load 3/RConn2
  Cable 3-3/RConn2 -- Cable 3-4/RConn2 -- Cable 2/RConn2 -- Cable 0/RConn2 -- Cable 3/LConn2 -- Cable 3-1/RConn2 -- Cable 3-2/RConn2
  Cable 3-2/RConn1 -- Cable 3-3/RConn1 -- Cable 3-4/RConn1 -- Cable 3/LConn1 -- Cable 0/RConn1 -- Current Sensor1/RConn2 -- Cable 3-1/RConn1
  Cable 3-2/LConn1 -- Battery 3/RConn1
  Cable 2-1/LConn1 -- Solar 2/RConn1
  Cable 2-1/LConn2 -- Solar 2/RConn2
  Cable 2-3/LConn1 -- Power load 2/RConn1
  Cable 2-2/LConn2 -- Battery 2/RConn2
  Cable 2-3/LConn2 -- Power load 2/RConn2
  Cable 2-3/RConn2 -- Cable 2/LConn2 -- Cable 1/RConn2 -- Cable 2-1/RConn2 -- Cable 2-2/RConn2
  Cable 2-2/RConn1 -- Current Sensor/RConn2 -- Cable 2/LConn1 -- Cable 2-1/RConn1 -- Cable 2-3/RConn1
  Cable 2-2/LConn1 -- Battery 2/RConn1
  Cable 1-1/LConn1 -- Solar 1/RConn1
  Cable 1-1/LConn2 -- Solar 1/RConn2
  Cable 1-3/LConn1 -- Power load 1/RConn1
  Cable 1-2/LConn2 -- Battery 1/RConn2
  Cable 1-3/LConn2 -- Power load 1/RConn2
  Cable 1-3/RConn2 -- Cable 1/LConn2 -- Cable 5/RConn2 -- Cable 1-1/RConn2 -- Cable 1-2/RConn2
  Cable 1-2/RConn1 -- Cable 1-3/RConn1 -- Cable 5/RConn1 -- Cable 1/LConn1 -- Cable 1-1/RConn1
  Cable 1-2/LConn1 -- Battery 1/RConn1
  Cable 4-1/LConn1 -- Solar 4/RConn1
  Cable 4-1/LConn2 -- Solar 4/RConn2
  Cable 4-3/LConn1 -- Power load 4/RConn1
  Cable 4-2/LConn2 -- Battery 4/RConn2
  Cable 4-3/LConn2 -- Power load 4/RConn2
  Cable 4-3/RConn2 -- Cable 4/LConn2 -- Cable 3/RConn2 -- Cable 4-1/RConn2 -- Cable 4-2/RConn2
  Cable 4-2/RConn1 -- Current Sensor2/RConn2 -- Cable 4/LConn1 -- Cable 4-1/RConn1 -- Cable 4-3/RConn1
  Cable 4-2/LConn1 -- Battery 4/RConn1
  Cable 5-1/LConn1 -- Solar 5/RConn1
  Cable 5-1/LConn2 -- Solar 5/RConn2
  Cable 5-3/LConn1 -- Power load 5/RConn1
  Cable 5-2/LConn2 -- Battery 5/RConn2
  Cable 5-3/LConn2 -- Power load 5/RConn2
  Cable 5-3/RConn2 -- Cable 4/RConn2 -- Cable 6/RConn2 -- Cable 5-1/RConn2 -- Cable 5-2/RConn2
  Cable 5-2/RConn1 -- Cable 6/RConn1 -- Current Sensor3/RConn2 -- Cable 5-1/RConn1 -- Cable 5-3/RConn1
  Cable 5-2/LConn1 -- Battery 5/RConn1
  Cable 5/LConn1 -- Wind 1/RConn1
  Cable 5/LConn2 -- Wind 1/RConn2
  Cable 3/RConn1 -- Current Sensor2/LConn1
  Cable 0/LConn2 -- Utility grid/RConn2
  Utility grid/RConn1 -- Cable 0/LConn1
  Cable 3-4/LConn2 -- EV charging/RConn2
  Cable 3-4/LConn1 -- EV charging/RConn1
  Current Sensor/RConn1 -- PS-Simulink Converter2/LConn1
  Current Sensor1/RConn1 -- PS-Simulink Converter/LConn1
  Current Sensor2/RConn1 -- PS-Simulink Converter1/LConn1
  Current Sensor3/LConn1 -- Cable 4/RConn1
  Current Sensor3/RConn1 -- PS-Simulink Converter3/LConn1
  Wind 2/RConn1 -- Cable 6/LConn1
  Wind 2/RConn2 -- Cable 6/LConn2

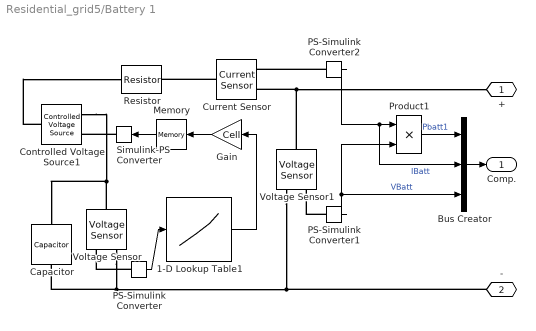
== system Residential_grid5/Battery 1 ==
  1-D Lookup Table1 : Lookup_n-D  NumberOfTableDimensions=1  BreakpointsForDimension1=[0;0.0001;0.00025000000000000001;0.00040000000000000002;0.0007000000000000001;0.001;0.0015;0.0023;0.0040000000000000001;0.0060000000000000001;0.007000000000000001;0.0080000000000000002;0.0089999999999999993;0.0094999999999999998;0.0097999999999999997;0.0099500000000000005;0.01]  Table=[0;1;2.7000000000000002;2.9500000000000002;3.1000000000000001;3.2000000000000002;3.2400000000000002;3.2599999999999998;3.2799999999999998;3.2999999999999998;3.3399999999999999;3.3500000000000001;3.3700000000000001;3.3900000000000001;3.4500000000000002;3.6000000000000001;3.8000000000000003]  InternalRulePriority=Speed  RndMeth=Simplest
  Bus Creator : BusCreator  Inputs=3
  Capacitor : fl_lib/Electrical/Electrical Elements/Capacitor  c=3.6e5*C_batt F  r=0 Ohm  g=0 1/Ohm  i_specify=off  i_priority=None  i=0 A  i_nominal_specify=off  i_nominal_value=1  i_nominal_unit=A  v_specify=off  v_priority=None  v=0 V  v_nominal_specify=off  v_nominal_value=1  v_nominal_unit=V  vc_specify=on  vc_priority=High  vc=SOC_Initial/10000 V  vc_nominal_specify=off  vc_nominal_value=1  vc_nominal_unit=V
  Controlled Voltage Source1 : fl_lib/Electrical/Electrical Sources/Controlled Voltage Source
  Current Sensor : fl_lib/Electrical/Electrical Sensors/Current Sensor
  Gain : Gain  Gain=Cell
  Memory : Memory
  PS-Simulink Converter : nesl_utility/PS-Simulink Converter  PhysicalDomain=network_engine_domain  SubClassName=ps_output  LeftPortType=input  RightPortType=output  PseudoPeriodic=off  Frequencies=[]  VectorFormat=inherit  Unit=inherit  AffineConversion=off
  PS-Simulink Converter1 : nesl_utility/PS-Simulink Converter  PhysicalDomain=network_engine_domain  SubClassName=ps_output  LeftPortType=input  RightPortType=output  PseudoPeriodic=off  Frequencies=[]  VectorFormat=inherit  Unit=inherit  AffineConversion=off
  PS-Simulink Converter2 : nesl_utility/PS-Simulink Converter  PhysicalDomain=network_engine_domain  SubClassName=ps_output  LeftPortType=input  RightPortType=output  PseudoPeriodic=off  Frequencies=[]  VectorFormat=inherit  Unit=inherit  AffineConversion=off
  Product1 : Product
  Resistor : fl_lib/Electrical/Electrical Elements/Resistor  R=1e-3*R_int*Cell/C_batt Ohm  i_specify=off  i_priority=None  i=0 A  i_nominal_specify=off  i_nominal_value=1  i_nominal_unit=A  v_specify=off  v_priority=None  v=0 V  v_nominal_specify=off  v_nominal_value=1  v_nominal_unit=V
  Simulink-PS Converter : nesl_utility/Simulink-PS Converter  PhysicalDomain=network_engine_domain  SubClassName=ps_input  LeftPortType=input  RightPortType=output  PseudoPeriodic=off  Frequencies=[]  NoiseDistribution=none  NoiseParameters=[]  Unit=1  AffineConversion=off  FilteringAndDerivatives=provide  SimscapeFilterOrder=1  InputFilterTimeConstant=0.001  UdotUserProvided=0
  Voltage Sensor : fl_lib/Electrical/Electrical Sensors/Voltage Sensor
  Voltage Sensor1 : fl_lib/Electrical/Electrical Sensors/Voltage Sensor
  + : PMIOPort  Side=Right
  - : PMIOPort  Port=2  Side=Right
  Comp. : Outport
  wires:
  PS-Simulink Converter2/1 -> Product1/1, Bus Creator/2  "IBatt"
  PS-Simulink Converter1/1 -> Bus Creator/3, Product1/2  "VBatt"
  Product1/1 -> Bus Creator/1  "Pbatt1"
  Bus Creator/1 -> Comp./1
  PS-Simulink Converter/1 -> 1-D Lookup Table1/1
  Memory/1 -> Simulink-PS Converter/1
  Gain/1 -> Memory/1
  1-D Lookup Table1/1 -> Gain/1
  connections:
  Voltage Sensor/LConn1 -- Controlled Voltage Source1/RConn2 -- Capacitor/LConn1
  Capacitor/RConn1 -- Voltage Sensor/RConn2 -- -/RConn1 -- Voltage Sensor1/RConn2
  Voltage Sensor1/LConn1 -- +/RConn1 -- Current Sensor/RConn2
  Current Sensor/LConn1 -- Resistor/RConn1
  PS-Simulink Converter/LConn1 -- Voltage Sensor/RConn1
  Controlled Voltage Source1/LConn1 -- Resistor/LConn1
  PS-Simulink Converter1/LConn1 -- Voltage Sensor1/RConn1
  PS-Simulink Converter2/LConn1 -- Current Sensor/RConn1
  Simulink-PS Converter/RConn1 -- Controlled Voltage Source1/RConn1

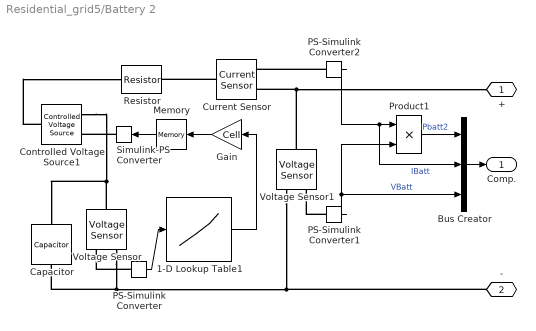
== system Residential_grid5/Battery 2 ==
  1-D Lookup Table1 : Lookup_n-D  NumberOfTableDimensions=1  BreakpointsForDimension1=[0;0.0001;0.00025000000000000001;0.00040000000000000002;0.0007000000000000001;0.001;0.0015;0.0023;0.0040000000000000001;0.0060000000000000001;0.007000000000000001;0.0080000000000000002;0.0089999999999999993;0.0094999999999999998;0.0097999999999999997;0.0099500000000000005;0.01]  Table=[0;1;2.7000000000000002;2.9500000000000002;3.1000000000000001;3.2000000000000002;3.2400000000000002;3.2599999999999998;3.2799999999999998;3.2999999999999998;3.3399999999999999;3.3500000000000001;3.3700000000000001;3.3900000000000001;3.4500000000000002;3.6000000000000001;3.8000000000000003]  InternalRulePriority=Speed  RndMeth=Simplest
  Bus Creator : BusCreator  Inputs=3
  Capacitor : fl_lib/Electrical/Electrical Elements/Capacitor  c=3.6e5*C_batt F  r=0 Ohm  g=0 1/Ohm  i_specify=off  i_priority=None  i=0 A  i_nominal_specify=off  i_nominal_value=1  i_nominal_unit=A  v_specify=off  v_priority=None  v=0 V  v_nominal_specify=off  v_nominal_value=1  v_nominal_unit=V  vc_specify=on  vc_priority=High  vc=SOC_Initial/10000 V  vc_nominal_specify=off  vc_nominal_value=1  vc_nominal_unit=V
  Controlled Voltage Source1 : fl_lib/Electrical/Electrical Sources/Controlled Voltage Source
  Current Sensor : fl_lib/Electrical/Electrical Sensors/Current Sensor
  Gain : Gain  Gain=Cell
  Memory : Memory
  PS-Simulink Converter : nesl_utility/PS-Simulink Converter  PhysicalDomain=network_engine_domain  SubClassName=ps_output  LeftPortType=input  RightPortType=output  PseudoPeriodic=off  Frequencies=[]  VectorFormat=inherit  Unit=inherit  AffineConversion=off
  PS-Simulink Converter1 : nesl_utility/PS-Simulink Converter  PhysicalDomain=network_engine_domain  SubClassName=ps_output  LeftPortType=input  RightPortType=output  PseudoPeriodic=off  Frequencies=[]  VectorFormat=inherit  Unit=inherit  AffineConversion=off
  PS-Simulink Converter2 : nesl_utility/PS-Simulink Converter  PhysicalDomain=network_engine_domain  SubClassName=ps_output  LeftPortType=input  RightPortType=output  PseudoPeriodic=off  Frequencies=[]  VectorFormat=inherit  Unit=inherit  AffineConversion=off
  Product1 : Product
  Resistor : fl_lib/Electrical/Electrical Elements/Resistor  R=1e-3*R_int*Cell/C_batt Ohm  i_specify=off  i_priority=None  i=0 A  i_nominal_specify=off  i_nominal_value=1  i_nominal_unit=A  v_specify=off  v_priority=None  v=0 V  v_nominal_specify=off  v_nominal_value=1  v_nominal_unit=V
  Simulink-PS Converter : nesl_utility/Simulink-PS Converter  PhysicalDomain=network_engine_domain  SubClassName=ps_input  LeftPortType=input  RightPortType=output  PseudoPeriodic=off  Frequencies=[]  NoiseDistribution=none  NoiseParameters=[]  Unit=1  AffineConversion=off  FilteringAndDerivatives=provide  SimscapeFilterOrder=1  InputFilterTimeConstant=0.001  UdotUserProvided=0
  Voltage Sensor : fl_lib/Electrical/Electrical Sensors/Voltage Sensor
  Voltage Sensor1 : fl_lib/Electrical/Electrical Sensors/Voltage Sensor
  + : PMIOPort  Side=Right
  - : PMIOPort  Port=2  Side=Right
  Comp. : Outport
  wires:
  PS-Simulink Converter2/1 -> Product1/1, Bus Creator/2  "IBatt"
  PS-Simulink Converter1/1 -> Bus Creator/3, Product1/2  "VBatt"
  Product1/1 -> Bus Creator/1  "Pbatt2"
  Bus Creator/1 -> Comp./1
  PS-Simulink Converter/1 -> 1-D Lookup Table1/1
  Memory/1 -> Simulink-PS Converter/1
  Gain/1 -> Memory/1
  1-D Lookup Table1/1 -> Gain/1
  connections:
  Voltage Sensor/LConn1 -- Controlled Voltage Source1/RConn2 -- Capacitor/LConn1
  Capacitor/RConn1 -- Voltage Sensor/RConn2 -- -/RConn1 -- Voltage Sensor1/RConn2
  Voltage Sensor1/LConn1 -- +/RConn1 -- Current Sensor/RConn2
  Current Sensor/LConn1 -- Resistor/RConn1
  PS-Simulink Converter/LConn1 -- Voltage Sensor/RConn1
  Controlled Voltage Source1/LConn1 -- Resistor/LConn1
  PS-Simulink Converter1/LConn1 -- Voltage Sensor1/RConn1
  PS-Simulink Converter2/LConn1 -- Current Sensor/RConn1
  Simulink-PS Converter/RConn1 -- Controlled Voltage Source1/RConn1

== system Residential_grid5/Battery 3 ==
  1-D Lookup Table1 : Lookup_n-D  NumberOfTableDimensions=1  BreakpointsForDimension1=[0;0.0001;0.00025000000000000001;0.00040000000000000002;0.0007000000000000001;0.001;0.0015;0.0023;0.0040000000000000001;0.0060000000000000001;0.007000000000000001;0.0080000000000000002;0.0089999999999999993;0.0094999999999999998;0.0097999999999999997;0.0099500000000000005;0.01]  Table=[0;1;2.7000000000000002;2.9500000000000002;3.1000000000000001;3.2000000000000002;3.2400000000000002;3.2599999999999998;3.2799999999999998;3.2999999999999998;3.3399999999999999;3.3500000000000001;3.3700000000000001;3.3900000000000001;3.4500000000000002;3.6000000000000001;3.8000000000000003]  InternalRulePriority=Speed  RndMeth=Simplest
  Bus Creator : BusCreator  Inputs=3
  Capacitor : fl_lib/Electrical/Electrical Elements/Capacitor  c=3.6e5*C_batt F  r=0 Ohm  g=0 1/Ohm  i_specify=off  i_priority=None  i=0 A  i_nominal_specify=off  i_nominal_value=1  i_nominal_unit=A  v_specify=off  v_priority=None  v=0 V  v_nominal_specify=off  v_nominal_value=1  v_nominal_unit=V  vc_specify=on  vc_priority=High  vc=SOC_Initial/10000 V  vc_nominal_specify=off  vc_nominal_value=1  vc_nominal_unit=V
  Controlled Voltage Source1 : fl_lib/Electrical/Electrical Sources/Controlled Voltage Source
  Current Sensor : fl_lib/Electrical/Electrical Sensors/Current Sensor
  Gain : Gain  Gain=Cell
  Memory : Memory
  PS-Simulink Converter : nesl_utility/PS-Simulink Converter  PhysicalDomain=network_engine_domain  SubClassName=ps_output  LeftPortType=input  RightPortType=output  PseudoPeriodic=off  Frequencies=[]  VectorFormat=inherit  Unit=inherit  AffineConversion=off
  PS-Simulink Converter1 : nesl_utility/PS-Simulink Converter  PhysicalDomain=network_engine_domain  SubClassName=ps_output  LeftPortType=input  RightPortType=output  PseudoPeriodic=off  Frequencies=[]  VectorFormat=inherit  Unit=inherit  AffineConversion=off
  PS-Simulink Converter2 : nesl_utility/PS-Simulink Converter  PhysicalDomain=network_engine_domain  SubClassName=ps_output  LeftPortType=input  RightPortType=output  PseudoPeriodic=off  Frequencies=[]  VectorFormat=inherit  Unit=inherit  AffineConversion=off
  Product1 : Product
  Resistor : fl_lib/Electrical/Electrical Elements/Resistor  R=1e-3*R_int*Cell/C_batt Ohm  i_specify=off  i_priority=None  i=0 A  i_nominal_specify=off  i_nominal_value=1  i_nominal_unit=A  v_specify=off  v_priority=None  v=0 V  v_nominal_specify=off  v_nominal_value=1  v_nominal_unit=V
  Simulink-PS Converter : nesl_utility/Simulink-PS Converter  PhysicalDomain=network_engine_domain  SubClassName=ps_input  LeftPortType=input  RightPortType=output  PseudoPeriodic=off  Frequencies=[]  NoiseDistribution=none  NoiseParameters=[]  Unit=1  AffineConversion=off  FilteringAndDerivatives=provide  SimscapeFilterOrder=1  InputFilterTimeConstant=0.001  UdotUserProvided=0
  Voltage Sensor : fl_lib/Electrical/Electrical Sensors/Voltage Sensor
  Voltage Sensor1 : fl_lib/Electrical/Electrical Sensors/Voltage Sensor
  + : PMIOPort  Side=Right
  - : PMIOPort  Port=2  Side=Right
  Comp. : Outport
  wires:
  PS-Simulink Converter2/1 -> Product1/1, Bus Creator/2  "IBatt"
  PS-Simulink Converter1/1 -> Bus Creator/3, Product1/2  "VBatt"
  Product1/1 -> Bus Creator/1  "Pbatt3"
  Bus Creator/1 -> Comp./1
  PS-Simulink Converter/1 -> 1-D Lookup Table1/1
  Memory/1 -> Simulink-PS Converter/1
  Gain/1 -> Memory/1
  1-D Lookup Table1/1 -> Gain/1
  connections:
  Voltage Sensor/LConn1 -- Controlled Voltage Source1/RConn2 -- Capacitor/LConn1
  Capacitor/RConn1 -- Voltage Sensor/RConn2 -- -/RConn1 -- Voltage Sensor1/RConn2
  Voltage Sensor1/LConn1 -- +/RConn1 -- Current Sensor/RConn2
  Current Sensor/LConn1 -- Resistor/RConn1
  PS-Simulink Converter/LConn1 -- Voltage Sensor/RConn1
  Controlled Voltage Source1/LConn1 -- Resistor/LConn1
  PS-Simulink Converter1/LConn1 -- Voltage Sensor1/RConn1
  PS-Simulink Converter2/LConn1 -- Current Sensor/RConn1
  Simulink-PS Converter/RConn1 -- Controlled Voltage Source1/RConn1

== system Residential_grid5/Battery 4 ==
  1-D Lookup Table1 : Lookup_n-D  NumberOfTableDimensions=1  BreakpointsForDimension1=[0;0.0001;0.00025000000000000001;0.00040000000000000002;0.0007000000000000001;0.001;0.0015;0.0023;0.0040000000000000001;0.0060000000000000001;0.007000000000000001;0.0080000000000000002;0.0089999999999999993;0.0094999999999999998;0.0097999999999999997;0.0099500000000000005;0.01]  Table=[0;1;2.7000000000000002;2.9500000000000002;3.1000000000000001;3.2000000000000002;3.2400000000000002;3.2599999999999998;3.2799999999999998;3.2999999999999998;3.3399999999999999;3.3500000000000001;3.3700000000000001;3.3900000000000001;3.4500000000000002;3.6000000000000001;3.8000000000000003]  InternalRulePriority=Speed  RndMeth=Simplest
  Bus Creator : BusCreator  Inputs=3
  Capacitor : fl_lib/Electrical/Electrical Elements/Capacitor  c=3.6e5*C_batt F  r=0 Ohm  g=0 1/Ohm  i_specify=off  i_priority=None  i=0 A  i_nominal_specify=off  i_nominal_value=1  i_nominal_unit=A  v_specify=off  v_priority=None  v=0 V  v_nominal_specify=off  v_nominal_value=1  v_nominal_unit=V  vc_specify=on  vc_priority=High  vc=SOC_Initial/10000 V  vc_nominal_specify=off  vc_nominal_value=1  vc_nominal_unit=V
  Controlled Voltage Source1 : fl_lib/Electrical/Electrical Sources/Controlled Voltage Source
  Current Sensor : fl_lib/Electrical/Electrical Sensors/Current Sensor
  Gain : Gain  Gain=Cell
  Memory : Memory
  PS-Simulink Converter : nesl_utility/PS-Simulink Converter  PhysicalDomain=network_engine_domain  SubClassName=ps_output  LeftPortType=input  RightPortType=output  PseudoPeriodic=off  Frequencies=[]  VectorFormat=inherit  Unit=inherit  AffineConversion=off
  PS-Simulink Converter1 : nesl_utility/PS-Simulink Converter  PhysicalDomain=network_engine_domain  SubClassName=ps_output  LeftPortType=input  RightPortType=output  PseudoPeriodic=off  Frequencies=[]  VectorFormat=inherit  Unit=inherit  AffineConversion=off
  PS-Simulink Converter2 : nesl_utility/PS-Simulink Converter  PhysicalDomain=network_engine_domain  SubClassName=ps_output  LeftPortType=input  RightPortType=output  PseudoPeriodic=off  Frequencies=[]  VectorFormat=inherit  Unit=inherit  AffineConversion=off
  Product1 : Product
  Resistor : fl_lib/Electrical/Electrical Elements/Resistor  R=1e-3*R_int*Cell/C_batt Ohm  i_specify=off  i_priority=None  i=0 A  i_nominal_specify=off  i_nominal_value=1  i_nominal_unit=A  v_specify=off  v_priority=None  v=0 V  v_nominal_specify=off  v_nominal_value=1  v_nominal_unit=V
  Simulink-PS Converter : nesl_utility/Simulink-PS Converter  PhysicalDomain=network_engine_domain  SubClassName=ps_input  LeftPortType=input  RightPortType=output  PseudoPeriodic=off  Frequencies=[]  NoiseDistribution=none  NoiseParameters=[]  Unit=1  AffineConversion=off  FilteringAndDerivatives=provide  SimscapeFilterOrder=1  InputFilterTimeConstant=0.001  UdotUserProvided=0
  Voltage Sensor : fl_lib/Electrical/Electrical Sensors/Voltage Sensor
  Voltage Sensor1 : fl_lib/Electrical/Electrical Sensors/Voltage Sensor
  + : PMIOPort  Side=Right
  - : PMIOPort  Port=2  Side=Right
  Comp. : Outport
  wires:
  PS-Simulink Converter2/1 -> Product1/1, Bus Creator/2  "IBatt"
  PS-Simulink Converter1/1 -> Bus Creator/3, Product1/2  "VBatt"
  Product1/1 -> Bus Creator/1  "Pbatt4"
  Bus Creator/1 -> Comp./1
  PS-Simulink Converter/1 -> 1-D Lookup Table1/1
  Memory/1 -> Simulink-PS Converter/1
  Gain/1 -> Memory/1
  1-D Lookup Table1/1 -> Gain/1
  connections:
  Voltage Sensor/LConn1 -- Controlled Voltage Source1/RConn2 -- Capacitor/LConn1
  Capacitor/RConn1 -- Voltage Sensor/RConn2 -- -/RConn1 -- Voltage Sensor1/RConn2
  Voltage Sensor1/LConn1 -- +/RConn1 -- Current Sensor/RConn2
  Current Sensor/LConn1 -- Resistor/RConn1
  PS-Simulink Converter/LConn1 -- Voltage Sensor/RConn1
  Controlled Voltage Source1/LConn1 -- Resistor/LConn1
  PS-Simulink Converter1/LConn1 -- Voltage Sensor1/RConn1
  PS-Simulink Converter2/LConn1 -- Current Sensor/RConn1
  Simulink-PS Converter/RConn1 -- Controlled Voltage Source1/RConn1
